simulink subsystem "GravityGradient"  (R2024b)
settings: Solver=VariableStepAuto  StartTime=0.0  StopTime=10.0  RelTol=1e-3
libraries: matrix_library x1
settings Model: Creator=marco  LastModifiedBy=ferru

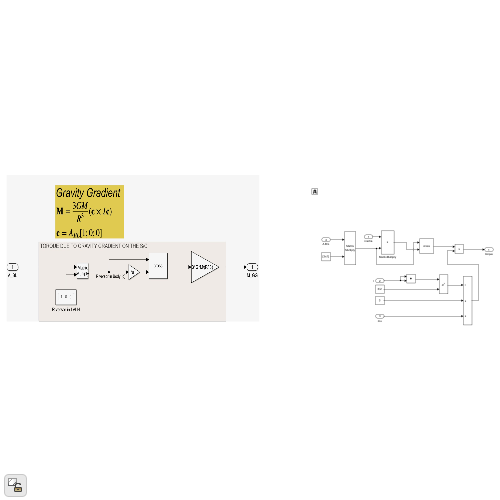
[thumbnail: Simulink's stored preview of the top-level diagram]
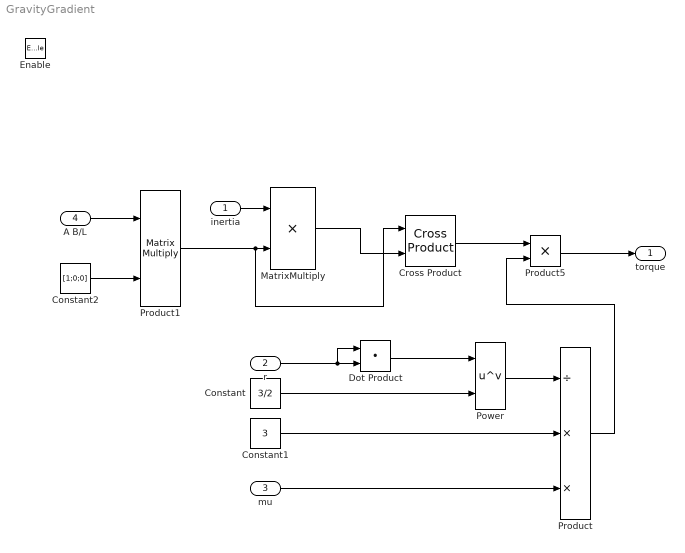
== system GravityGradient ==
  inertia : Inport
  r : Inport  Port=2
  mu : Inport  Port=3
  A B/L : Inport  Port=4
  Enable : EnablePort  StatesWhenEnabling=reset
  Constant : Constant  Value=3/2
  Constant1 : Constant  Value=3
  Constant2 : Constant  Value=[1;0;0]  VectorParams1D=off
  Cross Product : matrix_library/Cross Product
  Dot Product : DotProduct  OutDataTypeStr=Inherit: Inherit via internal rule
  MatrixMultiply : Product
  Power : Math  Operator=pow
  Product : Product  Inputs=/**
  Product1 : Product  Multiplication=Matrix(*)
  Product5 : Product
  torque : Outport  PortDimensions=[3, 1]
  wires:
  Constant/1 -> Power/2
  r/1 -> Dot Product/2, Dot Product/1
  Dot Product/1 -> Power/1
  Power/1 -> Product/1
  Constant1/1 -> Product/2
  mu/1 -> Product/3
  A B/L/1 -> Product1/1
  Constant2/1 -> Product1/2
  Product1/1 -> MatrixMultiply/2, Cross Product/1
  inertia/1 -> MatrixMultiply/1
  Cross Product/1 -> Product5/1
  Product/1 -> Product5/2
  Product5/1 -> torque/1
  MatrixMultiply/1 -> Cross Product/2
